simulink model "sldhdlc_mult_ConvergentRounding"  (R2026a)
settings: Solver=FixedStepDiscrete  StopTime=1000
InitFcn:
  | InputWL1 = 16;
  | InputFL1 = 12;
  | 
  | InputWL2 = 16;
  | InputFL2 = 5;
  | 
  | OutputWL = 20;
  | Delay = 1; % 1
  | ExtDelay = 0; %1
  | % Full-precision mult DT
  | MultWL = InputWL1 + InputWL2;
  | MultFL = InputFL1 + InputFL2;
  | IntBits = MultWL - MultFL; % integer bits
  | 
  | % Mult DT after rounding
  | OutputFL = OutputWL - IntBits;
libraries: simulink x2
settings Model: DataTypeOverride=Off  Creator=pnowodzi  LastModifiedBy=kkintali
settings OptimizationCC: ConditionallyExecuteInputs=off
settings DebuggingCC: AlgebraicLoopMsg=error  MergeDetectMultiDrivingBlocksExec=error  SingleTaskRateTransMsg=error  StrictBusMsg=ErrorOnBusTreatedAsVector
settings HardwareCC: ProdHWDeviceType=ASIC/FPGA->ASIC/FPGA  ProdEqTarget=off
settings ModelReferenceCC: PropagateSignalLabelsOutOfModel=on
settings ConfigComp: CovScope=ReferencedModels

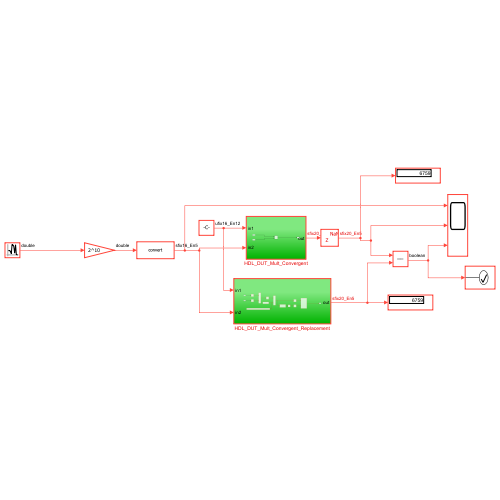
[thumbnail: Simulink's stored preview of the top-level diagram]
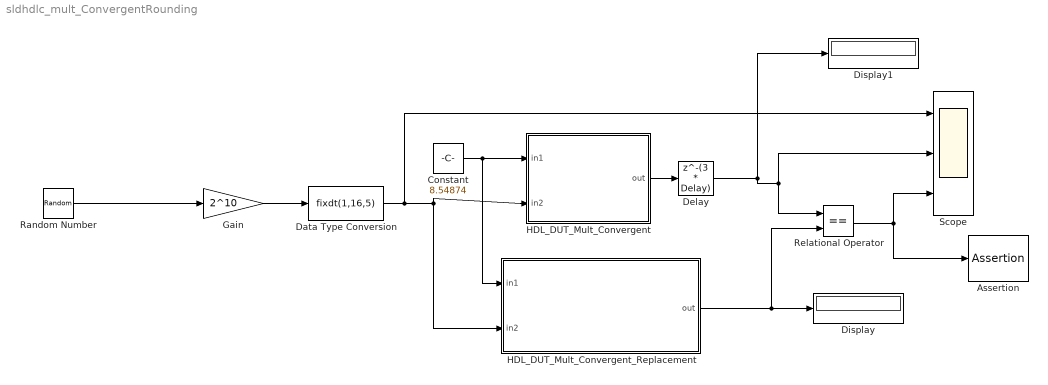
== system sldhdlc_mult_ConvergentRounding ==
  Assertion : Assertion
  Constant : Constant  Value=8.54874  OutDataTypeStr=fixdt(0,16,12)  SampleTime=-1
  Data Type Conversion : DataTypeConversion  OutDataTypeStr=fixdt(1,16,5)  SaturateOnIntegerOverflow=off  RndMeth=Floor
  Delay : Delay  DelayLength=(3 * Delay)
  Display : Display
  Display1 : Display
  Gain : Gain  Gain=2^10
  HDL_DUT_Mult_Convergent : Subsystem
  HDL_DUT_Mult_Convergent_Replacement : Subsystem
  Random Number : RandomNumber  SampleTime=1
  Relational Operator : RelationalOperator  Operator===  OutDataTypeStr=boolean  RndMeth=Simplest  InputSameDT=off
  Scope : Scope  NumInputPorts=3
      settings: TimeSpan=10  ActiveDisplayYMinimum=-1073.5508  ActiveDisplayYMaximum=1111.0195  DataLoggingSaveFormat=Array
  wires:
  Constant/1 -> HDL_DUT_Mult_Convergent_Replacement/1(in1), HDL_DUT_Mult_Convergent/1(in1)
  Random Number/1 -> Gain/1
  HDL_DUT_Mult_Convergent/1(out) -> Delay/1
  Data Type Conversion/1 -> Scope/1, HDL_DUT_Mult_Convergent_Replacement/2(in2), HDL_DUT_Mult_Convergent/2(in2)
  Gain/1 -> Data Type Conversion/1
  HDL_DUT_Mult_Convergent_Replacement/1(out) -> Relational Operator/2, Display/1
  Relational Operator/1 -> Assertion/1, Scope/3
  Delay/1 -> Relational Operator/1, Scope/2, Display1/1

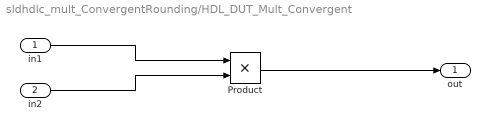
== system sldhdlc_mult_ConvergentRounding/HDL_DUT_Mult_Convergent ==
  in1 : Inport
  in2 : Inport  Port=2
  Product : Product  OutDataTypeStr=fixdt(1,20,5)  RndMeth=Convergent
  out : Outport  VectorParamsAs1DForOutWhenUnconnected=off
  wires:
  in1/1 -> Product/1
  in2/1 -> Product/2
  Product/1 -> out/1

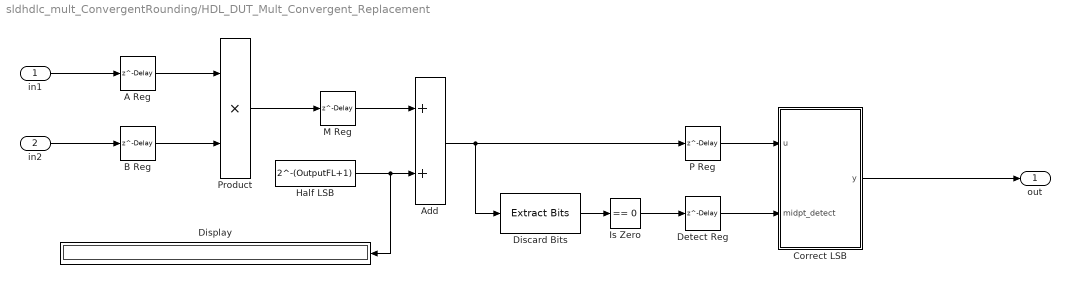
== system sldhdlc_mult_ConvergentRounding/HDL_DUT_Mult_Convergent_Replacement ==
  in1 : Inport
  in2 : Inport  Port=2
  A Reg : Delay  DelayLength=Delay
      settings: AttributesFormatString=ResetType : none
  Add : Sum  OutDataTypeStr=Inherit: Same as first input
  B Reg : Delay  DelayLength=Delay
      settings: AttributesFormatString=ResetType : none
  Correct LSB : MATLAB Function  TreatAsAtomicUnit=on
  Detect Reg : Delay  DelayLength=Delay
      settings: AttributesFormatString=ResetType : none
  Discard Bits : simulink/Logic and Bit Operations/Extract Bits  bitsToExtract=Range ending with least significant bit  numBits=MultWL-OutputWL  bitIdxRange=[0 7]  outScalingMode=Treat bit field as an integer
  Display : Display
      settings: Format=binary (Stored Integer)
  Half LSB : Constant  Value=2^-(OutputFL+1)  OutDataTypeStr=Inherit: Inherit via back propagation  SampleTime=-1
  Is Zero : simulink/Logic and Bit Operations/Compare To Constant  relop===  const=0  OutDataTypeStr=boolean
  M Reg : Delay  DelayLength=Delay
      settings: AttributesFormatString=ResetType : none
  P Reg : Delay  DelayLength=Delay
      settings: AttributesFormatString=ResetType : none
  Product : Product
  out : Outport  VectorParamsAs1DForOutWhenUnconnected=off
  wires:
  Is Zero/1 -> Detect Reg/1
  Correct LSB/1(y) -> out/1
  Detect Reg/1 -> Correct LSB/2(midpt_detect)
  P Reg/1 -> Correct LSB/1(u)
  Discard Bits/1 -> Is Zero/1
  Add/1 -> Discard Bits/1, P Reg/1
  M Reg/1 -> Add/1
  Half LSB/1 -> Display/1, Add/2
  B Reg/1 -> Product/2
  A Reg/1 -> Product/1
  in2/1 -> B Reg/1
  in1/1 -> A Reg/1
  Product/1 -> M Reg/1

== matlab function sldhdlc_mult_ConvergentRounding/HDL_DUT_Mult_Convergent_Replacement/Correct LSB ==
  settings: fimath=hdlfimath
  data: u input; midpt_detect input; y output; OutputWL parameter; OutputFL parameter
function y = fcn(u,midpt_detect,OutputWL,OutputFL)
%#codegen

NewLSB = u.WordLength - OutputWL + 1;
OutputDT = numerictype(1,OutputWL,OutputFL);

if midpt_detect
    % Round mid-point to even
    x = bitconcat(bitsliceget(u,u.WordLength,NewLSB+1),fi(0,0,1,0));
else
    x = bitsliceget(u,u.WordLength,NewLSB);
end

y = reinterpretcast(x,OutputDT);
